simulink library "propulsion_lib"  (R2018b)
settings: Solver=VariableStepAuto  StartTime=0.0  StopTime=10.0  RelTol=1e-3
undefined symbols (not defined in the file): prop, prop_map_fit, propDir, propInertia
libraries: $bdroot x3, axes_transformation_lib x2, unit_conversions_lib x1
settings Model: Creator=Ybeyer  LastModifiedBy=yannic
settings DebuggingCC: LibraryContextMissingDiagnostic=none
settings SFSimCC: SimUseLocalCustomCode=off
settings RTWCC: RTWUseLocalCustomCode=off
settings CodeAppCC: StateflowObjectComments=on

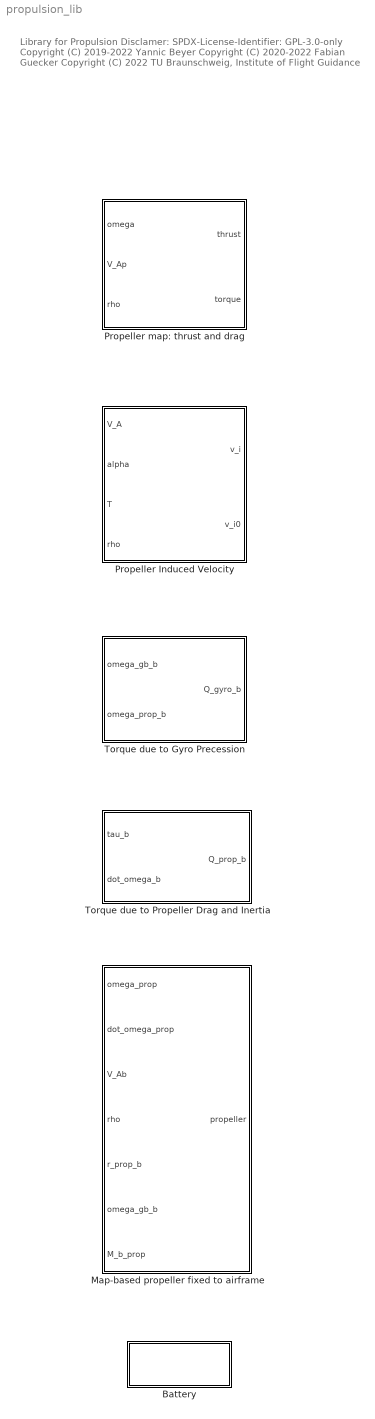
== system propulsion_lib ==
  note: Library for Propulsion
      |
      | Disclamer:
      | SPDX-License-Identifier: GPL-3.0-only
      |
      | Copyright (C) 2019-2022 Yannic Beyer
      | Copyright (C) 2020-2022 Fabian Guecker
      | Copyright (C) 2022 TU Braunschweig, Institute of Flight Guidance
  Battery : Subsystem
      settings: OpenFcn=battery_lib
  Map-based propeller fixed to airframe : Subsystem  mask{prop_map_fit=prop.map_fit, I_prop=propInertia, rotation_orientation=propDir(1)}
      mask prompts: prop_map_fit "Propeller map fit (see propMapFitCreate)"; I_prop "propeller moment of inertia, kg-m^2"; rotation_orientation "orientation of rotation (1: right, -1: left)"
      mask DialogControl DescGroupVar Prompt: Map-based propeller fixed to airframe
      mask DialogControl DescTextVar Prompt: This block computes the forces and moments generated by a propeller fixed to an airframe represented in body-fixed frame.
      mask DialogControl DescTextVar_copy Prompt: Moreover, other quantities like propeller thrust and torque are available in the output.
      mask DialogControl DescTextVar_copy_copy_copy_copy_copy_copy Prompt: Simplification: The angular velocity of the aircraft relative to the air or the earth is much smaller than the angular velocity of the propeller relative to the aircraft.
      mask DialogControl DescTextVar_copy_copy Prompt: (Add text here)
      mask DialogControl DescTextVar_copy_copy_copy Prompt: Inputs:
      mask DialogControl DescTextVar_copy_copy_copy_copy Prompt: scalar propeller angular velocity, in rad/s
      mask DialogControl DescTextVar_copy_copy_copy_copy_copy Prompt: scalar propeller angular acceleration, in rad/s
      mask DialogControl Control3 Prompt: airspeed vector of the center of mass represented in body-fixed frame, in m/s
      mask DialogControl Control4 Prompt: air density, in kg/m^3
      mask DialogControl Control5 Prompt: position vector of the propeller in body-fixed frame, in m
      mask DialogControl Control6 Prompt: angular velocity vector of the aircraft relative to the earth represented in body-fixed frame, in rad/s
      mask DialogControl Control7 Prompt: transformation matrix from propeller frame (x equals rotational axis) to body-fixed frame, in 1
      mask DialogControl Control8 Prompt: (Add text here)
      mask DialogControl Control9 Prompt: Outputs:
      mask DialogControl Control10 Prompt: bus including thrust, torque, resulting force and moment vector in body-fixed frame, airspeed vector in propeller frame
      mask DialogControl Container17 Prompt: Parameters
  Propeller Induced Velocity : Subsystem  mask{F=0.0507}
      mask prompts: F "surface of the propeller, m-2"
      mask DialogControl DescGroupVar Prompt: Propeller Induced Velocity
      mask DialogControl DescTextVar Prompt: Computation of the induced velocity of the propeller
      mask DialogControl Control3 Prompt: Inputs:
      mask DialogControl Control4 Prompt: V_A    absolute velocity of the propeller relative to the air, m/s
      mask DialogControl Control5 Prompt: alpha    angle between the rotor plane and the velocity vector relative to the air, rad
      mask DialogControl Control6 Prompt: T    thrust, N
      mask DialogControl Control7 Prompt: rho    air density, kg/m-3
      mask DialogControl Control8 Prompt: F    surface of the propeller, m-2
      mask DialogControl Control10 Prompt: Outputs:
      mask DialogControl Control11 Prompt: v_i    induced velocity of the propeller, m/s
      mask DialogControl Control12 Prompt: v_i0    induced velocity for V_A = 0, m/s
  Propeller map: thrust and drag : Subsystem  mask{prop_fit_map=prop_map_fit, rho_0=1.225}
      mask prompts: prop_fit_map "propeller map fit (see propMapFitCreate)"; rho_0 "reference air density, kg/m^3"
      mask DialogControl DescGroupVar Prompt: Propeller map: thrust and torque
      mask DialogControl DescTextVar Prompt: This block computes the thrust and torque generated by a propeller based on a map.
      mask DialogControl Control2 Prompt: The map depends on the angular velocity of the propeller as well as the airspeed perpendicular to the propeller rotational surface.
      mask DialogControl Control10 Prompt: (Add text here)
      mask DialogControl Control3 Prompt: Inputs:
      mask DialogControl Control4 Prompt: omega    (angular velocity of the propeller, 1/s)
      mask DialogControl Control5 Prompt: V_Ap     (airspeed in the propeller axes where x is the rotational axis, m/s)
      mask DialogControl Control6 Prompt: rho    (air density, kg/m^3)
      mask DialogControl Control11 Prompt: (Add text here)
      mask DialogControl Control7 Prompt: Outputs:
      mask DialogControl Control8 Prompt: T    (thrust, N)
      mask DialogControl Control9 Prompt: tau    (torque, Nm)
  Torque due to Gyro Precession : Subsystem  mask{J_prop=0.05}
      mask prompts: J_prop "Inertia (1xn) vector of n propellers, kg-m2"
      mask DialogControl DescGroupVar Prompt: Torque due to Gyro Precession
      mask DialogControl DescTextVar Prompt: Compute the torque generated by propellers with rotating rotation axis.
      mask DialogControl Control3 Prompt: Inputs:
      mask DialogControl Control4 Prompt: Angular velocity vector of aircraft relative to the earth in body-fixed axes (omega_gb_b), 1/s
      mask DialogControl Control5 Prompt: Angular velocity (3xn) matrix of n propellers in body-fixed axes (omega_prop_b), 1/s
      mask DialogControl Control7 Prompt: Outputs:
      mask DialogControl Control8 Prompt: Precesscion moment vector in body-fixed axes (Q_gyro_b), Nm
  Torque due to Propeller Drag and Inertia : Subsystem  mask{J_prop=0.05}
      mask prompts: J_prop "Propeller inertia (1xn) vector of n propellers, kg-m2"
      mask DialogControl DescGroupVar Prompt: Torque due to Propeller Drag and Inertia
      mask DialogControl DescTextVar Prompt: Compute the torque acting on the aircraft due to propeller drag and inertia.
      mask DialogControl Control3 Prompt: Inputs:
      mask DialogControl Control4 Prompt: Propeller torque (3xn) matrix of n propellers in body axes, Nm
      mask DialogControl Control5 Prompt: Propeller angular acceleration (3xn) matrix of n propellers in body axes, 1/s2
      mask DialogControl Control7 Prompt: Outputs:
      mask DialogControl Control8 Prompt: Moment vector in body axes, Nm

== system propulsion_lib/Battery ==

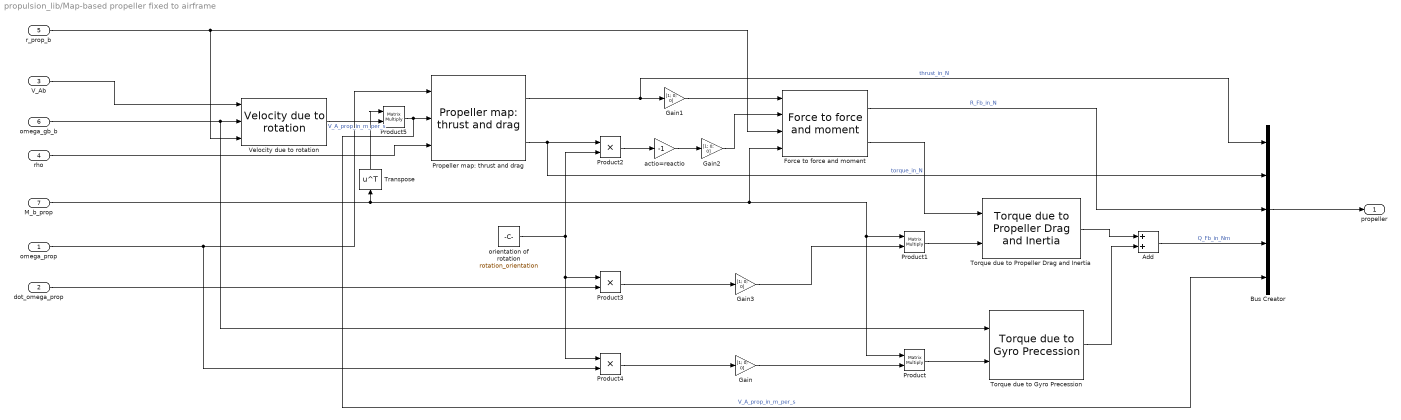
== system propulsion_lib/Map-based propeller fixed to airframe ==
  omega_prop : Inport
  dot_omega_prop : Inport  Port=2
  V_Ab : Inport  Port=3
  rho : Inport  Port=4
  r_prop_b : Inport  Port=5
  omega_gb_b : Inport  Port=6
  M_b_prop : Inport  Port=7
  Add : Sum
  Bus Creator : BusCreator  Inputs=5
  Force to force and moment : axes_transformation_lib/Force to force and moment  SystemSampleTime=-1
      settings: SourceProductName=LADAC
  Gain{,1..3} (4 alike) : Gain  Gain=[1; 0; 0]
  Product : Product  Multiplication=Matrix(*)
  Product1 : Product  Multiplication=Matrix(*)
  Product2 : Product
  Product3 : Product
  Product4 : Product
  Product5 : Product  Multiplication=Matrix(*)
  Propeller map: thrust and drag : $bdroot/Propeller map: thrust and drag  prop_fit_map=prop_map_fit  rho_0=1.225
  Torque due to Gyro Precession : $bdroot/Torque due to Gyro Precession  J_prop=I_prop
  Torque due to Propeller Drag and Inertia : $bdroot/Torque due to Propeller Drag and Inertia  J_prop=I_prop
  Transpose : Math  Operator=transpose  SaturateOnIntegerOverflow=on
  Velocity due to rotation : axes_transformation_lib/Velocity due to rotation  SystemSampleTime=-1
      settings: SourceProductName=LADAC
  actio=reactio : Gain  Gain=-1
  orientation of rotation : Constant  Value=rotation_orientation
  propeller : Outport
  wires:
  Torque due to Gyro Precession/1 -> Add/2
  Velocity due to rotation/1 -> Product5/2  "V_A_prop_in_m_per_s"
  Transpose/1 -> Product5/1
  Bus Creator/1 -> propeller/1
  Add/1 -> Bus Creator/4  "Q_Fb_in_Nm"
  V_Ab/1 -> Velocity due to rotation/1
  dot_omega_prop/1 -> Product3/2
  Gain3/1 -> Product1/2
  Force to force and moment/1 -> Bus Creator/3  "R_Fb_in_N"
  Force to force and moment/2 -> Torque due to Propeller Drag and Inertia/1
  Torque due to Propeller Drag and Inertia/1 -> Add/1
  Propeller map: thrust and drag/2 -> Product2/1, Bus Creator/2  "torque_in_N"
  Product/1 -> Torque due to Gyro Precession/2
  Product5/1 -> Bus Creator/5, Propeller map: thrust and drag/2  "V_A_prop_in_m_per_s"
  Propeller map: thrust and drag/1 -> Gain1/1, Bus Creator/1  "thrust_in_N"
  omega_gb_b/1 -> Velocity due to rotation/2, Torque due to Gyro Precession/1
  r_prop_b/1 -> Velocity due to rotation/3, Force to force and moment/3
  Product1/1 -> Torque due to Propeller Drag and Inertia/2
  omega_prop/1 -> Product4/2, Propeller map: thrust and drag/1
  M_b_prop/1 -> Force to force and moment/4, Product/1, Product1/1, Transpose/1
  rho/1 -> Propeller map: thrust and drag/3
  Gain/1 -> Product/2
  Gain1/1 -> Force to force and moment/1
  Gain2/1 -> Force to force and moment/2
  actio=reactio/1 -> Gain2/1
  Product2/1 -> actio=reactio/1
  Product3/1 -> Gain3/1
  orientation of rotation/1 -> Product2/2, Product4/1, Product3/1
  Product4/1 -> Gain/1

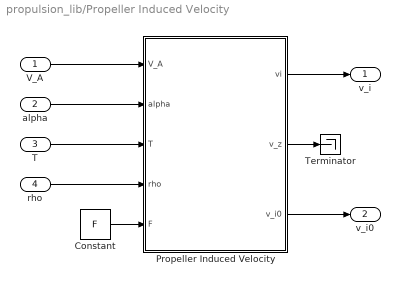
== system propulsion_lib/Propeller Induced Velocity ==
  V_A : Inport
  alpha : Inport  Port=2
  T : Inport  Port=3
  rho : Inport  Port=4
  Constant : Constant  Value=F
  Propeller Induced Velocity : MATLAB Function  TreatAsAtomicUnit=on
  Terminator : Terminator
  v_i : Outport
  v_i0 : Outport  Port=2
  wires:
  Constant/1 -> Propeller Induced Velocity/5(F)
  T/1 -> Propeller Induced Velocity/3(T)
  rho/1 -> Propeller Induced Velocity/4(rho)
  Propeller Induced Velocity/1(vi) -> v_i/1
  Propeller Induced Velocity/2(v_z) -> Terminator/1
  Propeller Induced Velocity/3(v_i0) -> v_i0/1
  alpha/1 -> Propeller Induced Velocity/2(alpha)
  V_A/1 -> Propeller Induced Velocity/1(V_A)

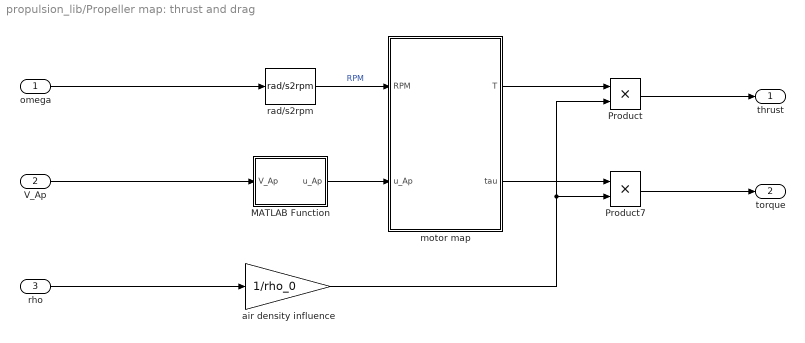
== system propulsion_lib/Propeller map: thrust and drag ==
  omega : Inport
  "V_Ap " : Inport  Port=2
  rho : Inport  Port=3
  MATLAB Function : MATLAB Function  TreatAsAtomicUnit=on
  Product : Product
  Product7 : Product
  air density influence : Gain  Gain=1/rho_0
  motor map : Subsystem
  rad/s2rpm : unit_conversions_lib/rad//s2rpm
      settings: SourceProductName=LADAC
  thrust : Outport
  torque : Outport  Port=2
  wires:
  omega/1 -> rad/s2rpm/1
  rho/1 -> air density influence/1
  "V_Ap "/1 -> MATLAB Function/1(V_Ap)
  Product7/1 -> torque/1
  rad/s2rpm/1 -> motor map/1(RPM)  "RPM"
  MATLAB Function/1(u_Ap) -> motor map/2(u_Ap)
  motor map/2(tau) -> Product7/1
  Product/1 -> thrust/1
  air density influence/1 -> Product7/2, Product/2
  motor map/1(T) -> Product/1

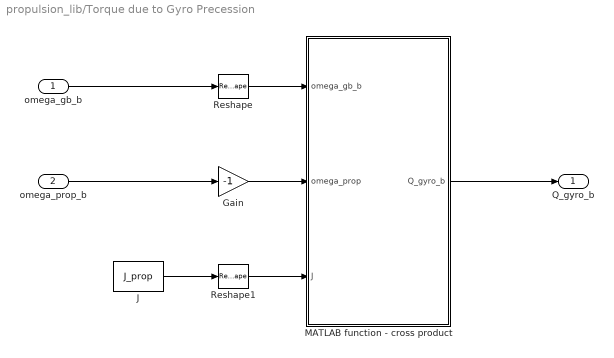
== system propulsion_lib/Torque due to Gyro Precession ==
  omega_gb_b : Inport
  omega_prop_b : Inport  Port=2
  Gain : Gain  Gain=-1
  J : Constant  Value=J_prop
  MATLAB function - cross product : MATLAB Function  TreatAsAtomicUnit=on
  Reshape : Reshape  OutputDimensionality=Column vector (2-D)
  Reshape1 : Reshape  OutputDimensionality=Row vector (2-D)
  Q_gyro_b : Outport
  wires:
  J/1 -> Reshape1/1
  omega_gb_b/1 -> Reshape/1
  Reshape/1 -> MATLAB function - cross product/1(omega_gb_b)
  omega_prop_b/1 -> Gain/1
  MATLAB function - cross product/1(Q_gyro_b) -> Q_gyro_b/1
  Reshape1/1 -> MATLAB function - cross product/3(J)
  Gain/1 -> MATLAB function - cross product/2(omega_prop)

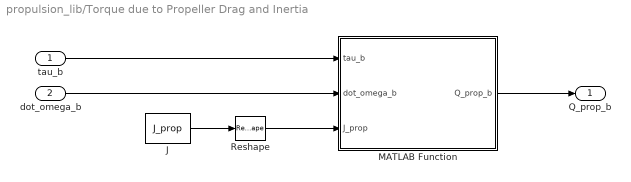
== system propulsion_lib/Torque due to Propeller Drag and Inertia ==
  tau_b : Inport
  dot_omega_b : Inport  Port=2
  J : Constant  Value=J_prop
  MATLAB Function : MATLAB Function  TreatAsAtomicUnit=on
  Reshape : Reshape  OutputDimensionality=Row vector (2-D)
  Q_prop_b : Outport
  wires:
  dot_omega_b/1 -> MATLAB Function/2(dot_omega_b)
  J/1 -> Reshape/1
  tau_b/1 -> MATLAB Function/1(tau_b)
  MATLAB Function/1(Q_prop_b) -> Q_prop_b/1
  Reshape/1 -> MATLAB Function/3(J_prop)

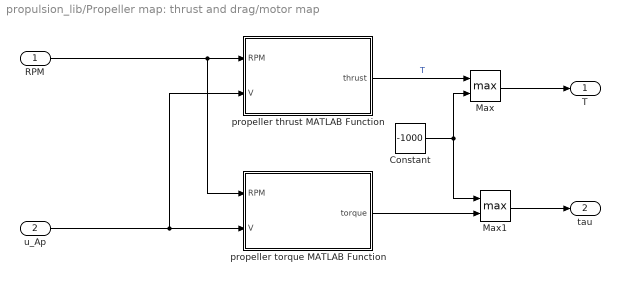
== system propulsion_lib/Propeller map: thrust and drag/motor map ==
  RPM : Inport
  u_Ap : Inport  Port=2
  Constant : Constant  Value=-1000
  Max : MinMax  Function=max  Inputs=2
  Max1 : MinMax  Function=max  Inputs=2
  propeller thrust MATLAB Function : MATLAB Function  TreatAsAtomicUnit=on
  propeller torque MATLAB Function : MATLAB Function  TreatAsAtomicUnit=on
  T : Outport
  tau : Outport  Port=2
  wires:
  propeller thrust MATLAB Function/1(thrust) -> Max/1  "T"
  RPM/1 -> propeller torque MATLAB Function/1(RPM), propeller thrust MATLAB Function/1(RPM)
  u_Ap/1 -> propeller torque MATLAB Function/2(V), propeller thrust MATLAB Function/2(V)
  propeller torque MATLAB Function/1(torque) -> Max1/2
  Max/1 -> T/1
  Max1/1 -> tau/1
  Constant/1 -> Max1/1, Max/2

== matlab function propulsion_lib/Propeller map: thrust and drag/MATLAB Function ==
  data: V_Ap input; u_Ap output
function u_Ap = fcn(V_Ap)
%#codegen

u_Ap = V_Ap(1,:);

== matlab function propulsion_lib/Propeller Induced Velocity/Propeller Induced Velocity ==
  data: V_A input; vi output; alpha input; T input; rho input; F input; v_z output; v_i0 output
function [ vi, v_z, v_i0 ] = fcn( V_A, alpha, T, rho, F ) %#codegen
    [ vi, v_z, v_i0 ] = propellerInducedVelocity( V_A, alpha, T, rho, F );
end

== matlab function propulsion_lib/Torque due to Propeller Drag and Inertia/MATLAB Function ==
  data: tau_b input; Q_prop_b output; dot_omega_b input; J_prop input
function Q_prop_b = fcn( tau_b, dot_omega_b, J_prop )
%#codegen

inertia_moment = dot_omega_b .* repmat( J_prop, 3, 1 );

Q_prop_b = sum( tau_b - inertia_moment, 2 );

== matlab function propulsion_lib/Propeller map: thrust and drag/motor map/propeller thrust MATLAB Function ==
  data: thrust output; RPM input; V input; prop_map_fit parameter
function thrust = propMapFitGetZ( RPM, V,  prop_map_fit)
thrust = propMapFitGetZ( prop_map_fit, RPM, V, 'thrust' );
end

== matlab function propulsion_lib/Propeller map: thrust and drag/motor map/propeller torque MATLAB Function ==
  data: torque output; RPM input; V input; prop_map_fit parameter
function torque = propMapFitGetZ( RPM, V,  prop_map_fit)
torque = propMapFitGetZ( prop_map_fit, RPM, V, 'torque' );
end

== matlab function propulsion_lib/Torque due to Gyro Precession/MATLAB function - cross product ==
  data: omega_gb_b input; Q_gyro_b output; omega_prop input; J input
function Q_gyro_b  = fcn(omega_gb_b,omega_prop,J)
%#codegen

% matrix generation
omega_gb_b = repmat( omega_gb_b, 1, length( omega_prop(1,:) ) );

% impulse computation
L_b_i = omega_prop .* repmat( J, 3, 1 );

% cross product
t1 = [2,3,1];
t2 = [3,1,2];
%C = A(:,t1).*B(:,t2)-A(:,t2).*B(:,t1);
Q_gyro_b_i = omega_gb_b(t1,:).*L_b_i(t2,:)-omega_gb_b(t2,:).*L_b_i(t1,:);

% sum of all propellers
Q_gyro_b = sum(Q_gyro_b_i,2);
